simulink model "adaptive_path_controller"  (R2026b)
settings: Solver=FixedStepDiscrete  FixedStep=0.05
settings Model: Creator=Ramakrishna  LastModifiedBy=Ramakrishna

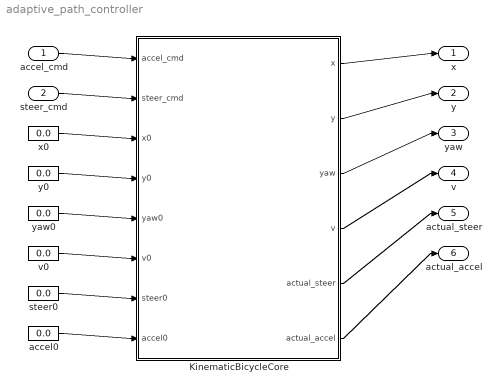
== system adaptive_path_controller ==
  accel_cmd : Inport
  steer_cmd : Inport  Port=2
  KinematicBicycleCore : MATLAB Function  TreatAsAtomicUnit=on
  accel0 : Constant  Value=0.0
  steer0 : Constant  Value=0.0
  v0 : Constant  Value=0.0
  x0 : Constant  Value=0.0
  y0 : Constant  Value=0.0
  yaw0 : Constant  Value=0.0
  x : Outport
  y : Outport  Port=2
  yaw : Outport  Port=3
  v : Outport  Port=4
  actual_steer : Outport  Port=5
  actual_accel : Outport  Port=6
  wires:
  accel_cmd/1 -> KinematicBicycleCore/1(accel_cmd)
  steer_cmd/1 -> KinematicBicycleCore/2(steer_cmd)
  x0/1 -> KinematicBicycleCore/3(x0)
  y0/1 -> KinematicBicycleCore/4(y0)
  yaw0/1 -> KinematicBicycleCore/5(yaw0)
  v0/1 -> KinematicBicycleCore/6(v0)
  steer0/1 -> KinematicBicycleCore/7(steer0)
  accel0/1 -> KinematicBicycleCore/8(accel0)
  KinematicBicycleCore/1(x) -> x/1
  KinematicBicycleCore/2(y) -> y/1
  KinematicBicycleCore/3(yaw) -> yaw/1
  KinematicBicycleCore/4(v) -> v/1
  KinematicBicycleCore/5(actual_steer) -> actual_steer/1
  KinematicBicycleCore/6(actual_accel) -> actual_accel/1

== matlab function adaptive_path_controller/KinematicBicycleCore ==
  data: x output; accel_cmd input; y output; steer_cmd input; x0 input; y0 input; yaw0 input; v0 input; steer0 input; accel0 input; yaw output; v output; actual_steer output; actual_accel output
function [x, y, yaw, v, actual_steer, actual_accel] = fcn(accel_cmd, steer_cmd, x0, y0, yaw0, v0, steer0, accel0)
% KINEMATIC BICYCLE MODEL CORE (ISO 8855)
% Exact discrete Forward Euler matching engine/simulation/vehicle.py
persistent px py pyaw pv p_steer p_accel initialized
if isempty(initialized)
    px = x0;
    py = y0;
    pyaw = yaw0;
    pv = v0;
    p_steer = steer0;
    p_accel = accel0;
    initialized = true;
end

% Parameters
wheelbase = 2.6;
dist_cg_to_rear = 1.3;
max_steer_rad = 0.60;
max_accel_m_s2 = 2.5;
max_decel_m_s2 = -6.5;
max_steer_rate_rad_s = 0.8;
max_jerk_m_s3 = 10.0;
dt = 0.05;

% 1. Saturation clamping
s_sat = max(-max_steer_rad, min(max_steer_rad, steer_cmd));
a_sat = max(max_decel_m_s2, min(max_accel_m_s2, accel_cmd));

% 2. Rate limiting
d_steer_max = max_steer_rate_rad_s * dt;
actual_steer = max(p_steer - d_steer_max, min(p_steer + d_steer_max, s_sat));
d_accel_max = max_jerk_m_s3 * dt;
actual_accel = max(p_accel - d_accel_max, min(p_accel + d_accel_max, a_sat));

% 3. Kinematic slip angle at CG
beta = atan((dist_cg_to_rear / wheelbase) * tan(actual_steer));

% 4. Derivatives
dx = pv * cos(pyaw + beta);
dy = pv * sin(pyaw + beta);
d_yaw = (pv / wheelbase) * cos(beta) * tan(actual_steer);

% 5. State output at step k
x = px;
y = py;
yaw = pyaw;
v = pv;

% 6. Forward Euler updates for next step k+1
px = px + dx * dt;
py = py + dy * dt;
pyaw = mod(pyaw + d_yaw * dt, 2 * pi);
pv = max(0.0, pv + actual_accel * dt);
p_steer = actual_steer;
p_accel = actual_accel;
